simulink model "PowerWindow_MIL"  (R2026b)
settings: Solver=FixedStepDiscrete  StopTime=20  FixedStep=0.01
undefined symbols (not defined in the file): InitPos, ObstacleActive, ObstaclePos, StallCurrent
libraries: simulink x2
settings Model: Creator=Vivekkumar Nandkishor  LastModifiedBy=Vivekkumar Nandkishor

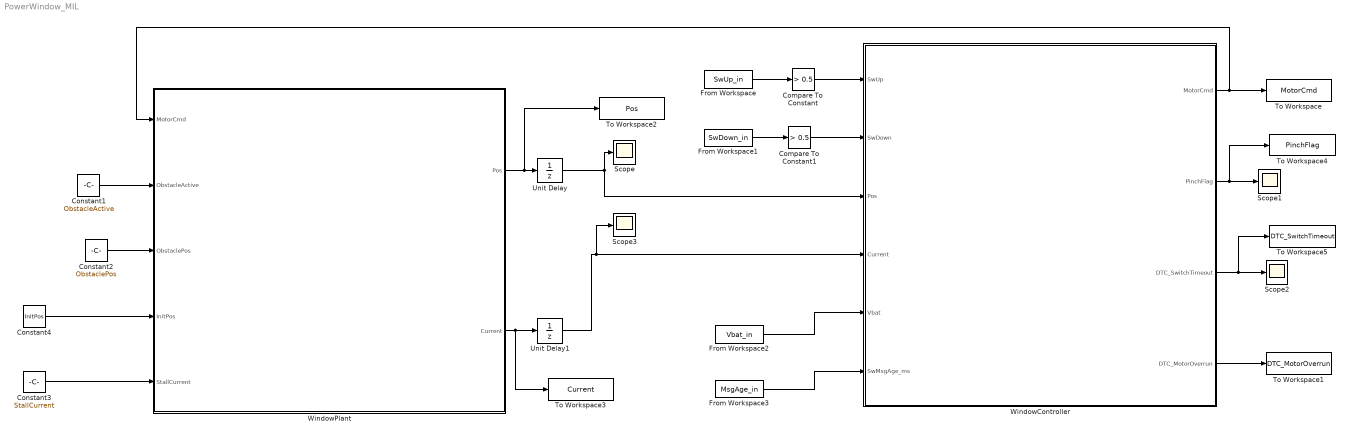
== system PowerWindow_MIL ==
  Compare To Constant : simulink/Logic and Bit Operations/Compare To Constant  relop=>  const=0.5  OutDataTypeStr=boolean
  Compare To Constant1 : simulink/Logic and Bit Operations/Compare To Constant  relop=>  const=0.5  OutDataTypeStr=boolean
  Constant1 : Constant  Value=ObstacleActive  SampleTime=0.01
  Constant2 : Constant  Value=ObstaclePos  SampleTime=0.01
  Constant3 : Constant  Value=StallCurrent  SampleTime=0.01
  Constant4 : Constant  Value=InitPos  SampleTime=0.01
  From Workspace : FromWorkspace  VariableName=SwUp_in  SampleTime=0.01  Interpolate=off  OutputAfterFinalValue=Holding final value
  From Workspace1 : FromWorkspace  VariableName=SwDown_in  SampleTime=0.01  Interpolate=off  OutputAfterFinalValue=Holding final value
  From Workspace2 : FromWorkspace  VariableName=Vbat_in  SampleTime=0.01  Interpolate=off  OutputAfterFinalValue=Holding final value
  From Workspace3 : FromWorkspace  VariableName=MsgAge_in  SampleTime=0.01  Interpolate=off  OutputAfterFinalValue=Holding final value
  Scope{,1..3} (4 alike) : Scope
      Scope settings: ActiveDisplayYMinimum=-2.1196430947666554  ActiveDisplayYMaximum=2.4643935408354127
      Scope1 settings: ActiveDisplayYMinimum=-0.44638566679687575  ActiveDisplayYMaximum=1.2287338839843751
      Scope2 settings: ActiveDisplayYMinimum=-1.2055441932692308  ActiveDisplayYMaximum=1.347018931730769  DataLoggingVariableName=ScopeData2
      Scope3 settings: ActiveDisplayYMinimum=-2.1196430947666554  ActiveDisplayYMaximum=2.4643935408354127  DataLoggingVariableName=ScopeData3
  To Workspace : ToWorkspace  VariableName=MotorCmd  SaveFormat=Timeseries  SampleTime=0.01
  To Workspace1 : ToWorkspace  VariableName=DTC_MotorOverrun  SaveFormat=Timeseries  SampleTime=0.01
  To Workspace2 : ToWorkspace  VariableName=Pos  SaveFormat=Timeseries  SampleTime=0.01
  To Workspace3 : ToWorkspace  VariableName=Current  SaveFormat=Timeseries  SampleTime=0.01
  To Workspace4 : ToWorkspace  VariableName=PinchFlag  SaveFormat=Timeseries  SampleTime=0.01
  To Workspace5 : ToWorkspace  VariableName=DTC_SwitchTimeout  SaveFormat=Timeseries  SampleTime=0.01
  Unit Delay : UnitDelay  InitialCondition=50  SampleTime=0.01
  Unit Delay1 : UnitDelay  SampleTime=0.01
  WindowController : Stateflow chart  TreatAsAtomicUnit=on
  WindowPlant : MATLAB Function  TreatAsAtomicUnit=on
  wires:
  Compare To Constant/1 -> WindowController/1(SwUp)
  WindowController/3(DTC_SwitchTimeout) -> To Workspace5/1, Scope2/1
  WindowController/2(PinchFlag) -> To Workspace4/1, Scope1/1
  WindowController/1(MotorCmd) -> WindowPlant/1(MotorCmd), To Workspace/1
  From Workspace2/1 -> WindowController/5(Vbat)
  Constant2/1 -> WindowPlant/3(ObstaclePos)
  Constant1/1 -> WindowPlant/2(ObstacleActive)
  Compare To Constant1/1 -> WindowController/2(SwDown)
  From Workspace3/1 -> WindowController/6(SwMsgAge_ms)
  WindowPlant/1(Pos) -> To Workspace2/1, Unit Delay/1
  WindowPlant/2(Current) -> To Workspace3/1, Unit Delay1/1
  Unit Delay1/1 -> WindowController/4(Current), Scope3/1
  Unit Delay/1 -> WindowController/3(Pos), Scope/1
  From Workspace/1 -> Compare To Constant/1
  From Workspace1/1 -> Compare To Constant1/1
  Constant3/1 -> WindowPlant/5(StallCurrent)
  WindowController/4(DTC_MotorOverrun) -> To Workspace1/1
  Constant4/1 -> WindowPlant/4(InitPos)

== matlab function PowerWindow_MIL/WindowPlant ==
  data: MotorCmd input; Pos output; ObstacleActive input; ObstaclePos input; InitPos input; Current output; StallCurrent input
function [Pos, Current] = WindowPlant(MotorCmd, ObstacleActive, ObstaclePos, InitPos, StallCurrent)
persistent p
if isempty(p)
    p = InitPos;
end

dt = 0.01;
speed = 25;
cmd = double(MotorCmd);
pNew = p + cmd * speed * dt;
blocked = false;

if cmd > 0 && ObstacleActive && p <= ObstaclePos && pNew >= ObstaclePos
    pNew = ObstaclePos;
    blocked = true;
end

if pNew >= 100
    pNew = 100;
    blocked = (cmd > 0);
elseif pNew <= 0
    pNew = 0;
    blocked = (cmd < 0);
end

if cmd == 0
    Current = 0;
elseif blocked
    Current = StallCurrent;
else
    Current = 2;
end

p = pNew;
Pos = p;
end

== stateflow chart PowerWindow_MIL/WindowController ==
  settings: updateMethod=DISCRETE  sampleTime=0.01
  state IDLE
    entry: MotorCmd =int8(0);
  state MOVING_UP
    entry: MotorCmd =int8(1);
  state WAIT_RELEASE
    entry: MotorCmd = int8(0);
  state PINCH_REVERSE
    entry: MotorCmd =int8(-1); PinchFlag = true;
  state MOVING_DOWN
    entry: MotorCmd =int8(-1);
  state ERROR
    entry: MotorCmd =int8(0);
  MOVING_UP -> IDLE [order 6] : [~SwUp || Pos >= 100] % REQ_03,REQ_04
  MOVING_UP -> IDLE [order 4] : [SwUp && SwDown] % REQ_11
  MOVING_UP -> IDLE [order 3] : [Vbat < 9 || Vbat > 16] %REQ_08
  (default) -> IDLE
  MOVING_DOWN -> IDLE [order 4] : [SwUp && SwDown] %REQ_11
  MOVING_DOWN -> IDLE [order 3] : [Vbat < 9 || Vbat > 16] %REQ_08
  IDLE -> MOVING_UP [order 2] : [SwUp && ~SwDown && Pos < 100 && Vbat >= 9 && Vbat <= 16 && SwMsgAge_ms <= 500]
  MOVING_UP -> PINCH_REVERSE [order 5] : [Current > 8 && Pos > 4 && Pos < 96]{PosAtPinch = Pos;} %REQ_05, REQ_07
  MOVING_UP -> ERROR [order 1] : [SwMsgAge_ms > 500]{DTC_SwitchTimeout = true;}%REQ_09
  MOVING_UP -> ERROR [order 2] : [after(8, sec)]{DTC_MotorOverrun = true;} %REQ_10
  MOVING_DOWN -> IDLE [order 5] : [~SwDown || Pos <= 0] %REQ_03,REQ_04
  IDLE -> MOVING_DOWN [order 3] : [SwDown && ~SwUp && Pos > 0 && Vbat >= 9 && Vbat <= 16 && SwMsgAge_ms <= 500]
  WAIT_RELEASE -> IDLE [order 2] : [~SwUp]{PinchFlag = false;}
  IDLE -> ERROR [order 1] : [SwMsgAge_ms > 500]{DTC_SwitchTimeout = true;} % REQ_09 CR_01
  ERROR -> IDLE : [SwMsgAge_ms <= 500 && ~SwUp && ~SwDown]{PinchFlag = false;}
  PINCH_REVERSE -> IDLE [order 3] : [Vbat < 9 || Vbat > 16] {PinchFlag = false;} %REQ_08
  PINCH_REVERSE -> WAIT_RELEASE [order 4] : [PosAtPinch - Pos >= 20 || Pos <= 0] % REQ_06
  WAIT_RELEASE -> ERROR [order 1] : [SwMsgAge_ms > 500]{DTC_SwitchTimeout = true;} % REQ_09 CR_01
  PINCH_REVERSE -> ERROR [order 2] : [after(8, sec)]{DTC_MotorOverrun = true;}
  PINCH_REVERSE -> ERROR [order 1] : [SwMsgAge_ms > 500]{DTC_SwitchTimeout = true;}
  MOVING_DOWN -> ERROR [order 1] : [SwMsgAge_ms > 500]{DTC_SwitchTimeout = true;} % REQ_09
  MOVING_DOWN -> ERROR [order 2] : [after(8, sec)]{DTC_MotorOverrun = true;} % REQ_10
  data: MotorCmd output int8; SwUp input boolean; SwDown input boolean; Pos input double; Current input double; Vbat input double; SwMsgAge_ms input double; PinchFlag output boolean; DTC_SwitchTimeout output boolean; DTC_MotorOverrun output boolean; PosAtPinch local double
